simulink model "Ahmad_Ro"  (R2025b)
settings: Solver=VariableStepAuto  StartTime=0.0  StopTime=10.0  RelTol=1e-3
undefined symbols (not defined in the file or in its folder): X, Y, Z
libraries: sm_lib x16, nesl_utility x5, robotcorelib x1, robotmaniplib x1
settings Model: Creator=Ahmad Hz  LastModifiedBy=Ahmad Hz
settings ExplorerConfigSet: InternalSimMechanicsExplorerSettings=|
  | <ExplorerConfiguration>
  | 
  |   <canonicalview>default</canonicalview>
  | 
  |   <TilePanel>
  |     <TileInfo>
  |       <Tiles Columns="1" Count="1" Height="498" Rows="1" Width="971">
  |         <Row Weight="1"/>
  |         <Column Weight="1"/>
  |         <Tile Height="1" Width="1" X="0" Y="0"/>
  |       </Tiles>
  |     </TileInfo>
  |     <SceneInfo>
  |       <SceneViewer>
  |         <IsThisViewStd>
  |           <IsStandardView>off</IsStandardView>
  |           <StandardViewName>Front</StandardViewName>
  |         </IsThisViewStd>
  |         <BGColor>
  |           <R>1</R>
  |           <G>1</G>
  |           <B>1</B>
  |           <A>1</A>
  |         </BGColor>
  |         <Camera>
  |           <DoPerspective>off</DoPerspective>
  |           <Position>
  |             <X>0.69878161416282247</X>
  |             <Y>-0.56958841515750935</Y>
  |             <Z>0.67013251417587816</Z>
  |           </Position>
  |           <Center>
  |             <X>0.088649099502656606</X>
  |             <Y>0.040544099502656611</Y>
  |             <Z>0.059999999515712263</Z>
  |           </Center>
  |           <Up>
  |             <X>-0.40824829046386313</X>
  |             <Y>0.40824829046386302</Y>
  |             <Z>0.81649658092772603</Z>
  |           </Up>
  |           <XLim>0.14683425317748552</XLim>
  |           <YLim>0.14683425317748552</YLim>
  |           <ViewLimDist>0.01</ViewLimDist>
  |         </Camera>
  |       </SceneViewer>
  |     </SceneInfo>
  |   </TilePanel>
  | 
  |   <MechEditorPanel>
  |     <GfxPanelCameraMap/>
  |     <Cameras/>
  |     <VideoCreator>
  |       <IncludeTiles>All</IncludeTiles>
  |       <IncludeTime>on</IncludeTime>
  |       <IncludeWorldFrame>off</IncludeWorldFrame>
  |       <PlaybackSpeedRatio>1</PlaybackSpeedRatio>
  |       <FrameRate>30</FrameRate>
  |       <FrameSize>auto</FrameSize>
  |       <VideoFormat>MotionJPEGAVI</VideoFormat>
  |     </VideoCreator>
  |   </MechEditorPanel>
  | 
  |   <PlaybackSettings>
  |     <PlaybackSpeedFactor>1</PlaybackSpeedFactor>
  |   </PlaybackSettings>
  | 
  | </ExplorerConfiguration>

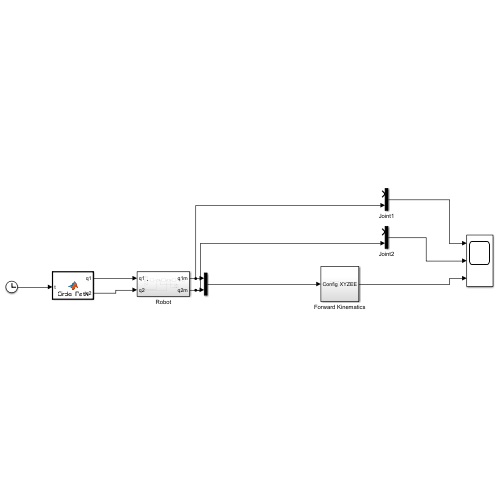
[thumbnail: Simulink's stored preview of the top-level diagram]
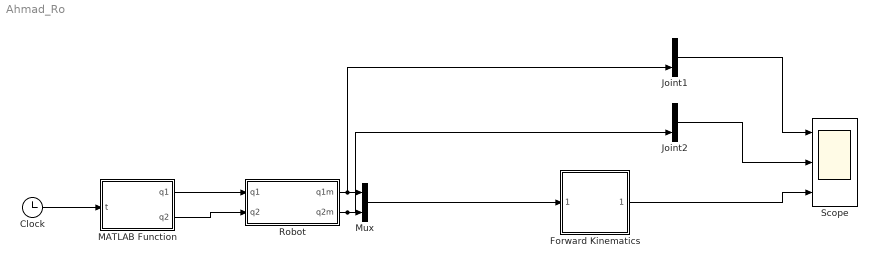
== system Ahmad_Ro ==
  Clock : Clock
  Forward Kinematics : Subsystem
  Joint1 : Mux  Inputs=2
  Joint2 : Mux  Inputs=2
  MATLAB Function : MATLAB Function  TreatAsAtomicUnit=on
  Mux : Mux  Inputs=2
  Robot : Subsystem
  Scope : Scope  NumInputPorts=3
      settings: ActiveDisplayYMinimum=-2.7504115188527223  ActiveDisplayYMaximum=3.3779479158130368
  wires:
  Robot/1(q1m) -> Joint1/2, Mux/1
  Robot/2(q2m) -> Joint2/2, Mux/2
  Joint1/1 -> Scope/1
  Joint2/1 -> Scope/2
  Mux/1 -> Forward Kinematics/1(Config)
  Forward Kinematics/1(XYZEE) -> Scope/3
  MATLAB Function/1(q1) -> Robot/1(q1)
  MATLAB Function/2(q2) -> Robot/2(q2)
  Clock/1 -> MATLAB Function/1(t)

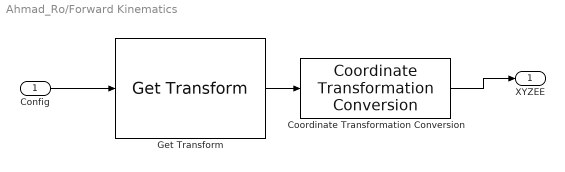
== system Ahmad_Ro/Forward Kinematics ==
  Config : Inport
  Coordinate Transformation Conversion : robotcorelib/Coordinate Transformation Conversion  InputRepresentation=Homogeneous Transformation  InputEulerSequence=ZYX  ShowTrVecInputPort=on  OutputRepresentation=Translation Vector  OutputEulerSequence=ZYX  ShowTrVecOutputPort=on  SimulateUsing=Interpreted execution
  Get Transform : robotmaniplib/Get Transform  RigidBodyTree=twoJointRigidBodyTree  SourceBody=tool  TargetBody=base  SimulateUsing=Interpreted execution
  XYZEE : Outport
  wires:
  Get Transform/1 -> Coordinate Transformation Conversion/1
  Coordinate Transformation Conversion/1 -> XYZEE/1
  Config/1 -> Get Transform/1

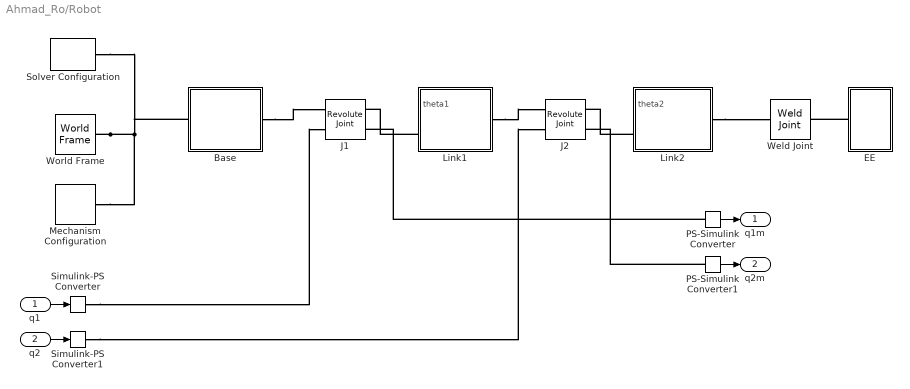
== system Ahmad_Ro/Robot ==
  q1 : Inport
  q2 : Inport  Port=2
  Base : Subsystem
  EE : Subsystem
  J1 : sm_lib/Joints/Revolute Joint  JointMode=Normal  CompositeWrenchDir=FollowerOnBase  CompositeWrenchFrame=BaseFrame  SenseConstraintForce=off  SenseConstraintTorque=off  SenseTotalForce=off  SenseTotalTorque=off  PositionTargetSpecify=off  PositionTargetPriority=High  PositionTargetValue=0  PositionTargetValueUnits=deg  VelocityTargetSpecify=off  VelocityTargetPriority=High  VelocityTargetValue=0  VelocityTargetValueUnits=deg/s  EquilibriumPosition=0  EquilibriumPositionUnits=deg  SpringStiffness=0  SpringStiffnessUnits=N*m/deg  DampingCoefficient=0  DampingCoefficientUnits=N*m/(deg/s)  LowerLimitSpecify=on  LowerLimitBound=-90  LowerLimitBoundUnits=deg  LowerLimitStiffness=1e4  LowerLimitStiffnessUnits=N*m/deg  LowerLimitDamping=10  LowerLimitDampingUnits=N*m/(deg/s)  LowerLimitTransitionRegionWidth=0.1  LowerLimitTransitionRegionWidthUnits=deg  UpperLimitSpecify=on  UpperLimitBound=90  UpperLimitBoundUnits=deg  UpperLimitStiffness=1e4  UpperLimitStiffnessUnits=N*m/deg  UpperLimitDamping=10  UpperLimitDampingUnits=N*m/(deg/s)  UpperLimitTransitionRegionWidth=0.1  UpperLimitTransitionRegionWidthUnits=deg  TorqueActuationMode=ComputedTorque  MotionActuationMode=InputMotion  SensePosition=on  SenseVelocity=off  SenseAcceleration=off  SenseTorqueForce=off  SenseLowerLimitTorqueForce=off  SenseUpperLimitTorqueForce=off
  J2 : sm_lib/Joints/Revolute Joint  JointMode=Normal  CompositeWrenchDir=FollowerOnBase  CompositeWrenchFrame=BaseFrame  SenseConstraintForce=off  SenseConstraintTorque=off  SenseTotalForce=off  SenseTotalTorque=off  PositionTargetSpecify=off  PositionTargetPriority=High  PositionTargetValue=0  PositionTargetValueUnits=deg  VelocityTargetSpecify=off  VelocityTargetPriority=High  VelocityTargetValue=0  VelocityTargetValueUnits=deg/s  EquilibriumPosition=0  EquilibriumPositionUnits=deg  SpringStiffness=0  SpringStiffnessUnits=N*m/deg  DampingCoefficient=0  DampingCoefficientUnits=N*m/(deg/s)  LowerLimitSpecify=on  LowerLimitBound=-60  LowerLimitBoundUnits=deg  LowerLimitStiffness=1e4  LowerLimitStiffnessUnits=N*m/deg  LowerLimitDamping=10  LowerLimitDampingUnits=N*m/(deg/s)  LowerLimitTransitionRegionWidth=0.1  LowerLimitTransitionRegionWidthUnits=deg  UpperLimitSpecify=on  UpperLimitBound=60  UpperLimitBoundUnits=deg  UpperLimitStiffness=1e4  UpperLimitStiffnessUnits=N*m/deg  UpperLimitDamping=10  UpperLimitDampingUnits=N*m/(deg/s)  UpperLimitTransitionRegionWidth=0.1  UpperLimitTransitionRegionWidthUnits=deg  TorqueActuationMode=ComputedTorque  MotionActuationMode=InputMotion  SensePosition=on  SenseVelocity=off  SenseAcceleration=off  SenseTorqueForce=off  SenseLowerLimitTorqueForce=off  SenseUpperLimitTorqueForce=off
  Link1 : Subsystem
  Link2 : Subsystem
  Mechanism Configuration : sm_lib/Utilities/Mechanism Configuration  UniformGravity=Constant  GravityVector=[0 0 -9.80665]  GravityVectorUnits=m/s^2  LinearizationDelta=0.001  JointModeTransitionNonlinearIterations=2
  PS-Simulink Converter : nesl_utility/PS-Simulink Converter  PhysicalDomain=network_engine_domain  SubClassName=ps_output  LeftPortType=input  RightPortType=output  PseudoPeriodic=off  Frequencies=[]  VectorFormat=inherit  Unit=inherit  AffineConversion=off
  PS-Simulink Converter1 : nesl_utility/PS-Simulink Converter  PhysicalDomain=network_engine_domain  SubClassName=ps_output  LeftPortType=input  RightPortType=output  PseudoPeriodic=off  Frequencies=[]  VectorFormat=inherit  Unit=inherit  AffineConversion=off
  Simulink-PS Converter : nesl_utility/Simulink-PS Converter  PhysicalDomain=network_engine_domain  SubClassName=ps_input  LeftPortType=input  RightPortType=output  PseudoPeriodic=off  Frequencies=[]  NoiseDistribution=none  NoiseParameters=[]  Unit=rad  AffineConversion=off  FilteringAndDerivatives=filter  SimscapeFilterOrder=2  InputFilterTimeConstant=0.001  UdotUserProvided=0
  Simulink-PS Converter1 : nesl_utility/Simulink-PS Converter  PhysicalDomain=network_engine_domain  SubClassName=ps_input  LeftPortType=input  RightPortType=output  PseudoPeriodic=off  Frequencies=[]  NoiseDistribution=none  NoiseParameters=[]  Unit=rad  AffineConversion=off  FilteringAndDerivatives=filter  SimscapeFilterOrder=2  InputFilterTimeConstant=0.001  UdotUserProvided=0
  Solver Configuration : nesl_utility/Solver Configuration  PhysicalDomain=network_engine_domain  SubClassName=solver  LeftPortType=input  RightPortType=generic  Tones=[]  Harmonics=[]  SimulateNoise=off  Profile=off  UseLocalSampling=off  EnableSwitchedLinearOptims=on  FrequencyDomain=off  UseCCode=off  RelTol=0.001  AbsTol=0.001  MinStep=1e-09  ToWorkspace=off  RevertToSquareIcSolve=off  NumHomotopyIterations=100  PhasorMode=off  PhasorModeNumHarmonics=1  ConsistencySolver=NEWTON_XTOL_AFTER_FTOL  IndexReductionMethod=DerivativeReplacement  DoDC=off  ResidualTolerance=1e-09  ConsistencyTolSource=GLOBAL  ConsistencyAbsTol=0.001  ConsistencyRelTol=0.001  ConsistencyTolFactor=0.001  UseLocalSolver=off  LocalSolverChoice=NE_BACKWARD_EULER_ADVANCER  ResolveIndetEquations=on  FunctionEvalNumThread=1  LocalSolverSampleTime=0.001  DoFixedCost=off  MaxNonlinIter=3  MaxModeIter=2  ComputeImpulses=off  ImpulseIterations=2  LinearAlgebra=auto  LinearAlgebraNumThread=0  EquationFormulation=NE_TIME_EF  DelaysMemoryBudget=1024  AutomaticFiltering=on  FilteringTimeConstant=0.001  PartitionStorageMethod=AS_NEEDED  PartitionMemoryBudget=1024  PartitionMethod=ROBUST  MultibodyUseLocalSolver=off  MultibodyLocalSolverChoice=ODE1  MultibodyLocalSolverSampleTime=0.001
  Weld Joint : sm_lib/Joints/Weld Joint  JointMode=Normal  CompositeWrenchDir=FollowerOnBase  CompositeWrenchFrame=BaseFrame  SenseConstraintForce=off  SenseConstraintTorque=off  SenseTotalForce=off  SenseTotalTorque=off
  World Frame : sm_lib/Frames and Transforms/World Frame
  q1m : Outport
  q2m : Outport  Port=2
  wires:
  q2/1 -> Simulink-PS Converter1/1
  PS-Simulink Converter/1 -> q1m/1
  q1/1 -> Simulink-PS Converter/1
  PS-Simulink Converter1/1 -> q2m/1
  connections:
  Link1/LConn1 -- J1/RConn1
  EE/LConn1 -- Weld Joint/RConn1
  World Frame/RConn1 -- Solver Configuration/RConn1 -- Base/LConn1 -- Mechanism Configuration/RConn1
  PS-Simulink Converter1/LConn1 -- J2/RConn2
  Simulink-PS Converter1/RConn1 -- J2/LConn2
  PS-Simulink Converter/LConn1 -- J1/RConn2
  Link1/RConn1 -- J2/LConn1
  Base/RConn1 -- J1/LConn1
  Link2/RConn1 -- Weld Joint/LConn1
  Link2/LConn1 -- J2/RConn1
  Simulink-PS Converter/RConn1 -- J1/LConn2

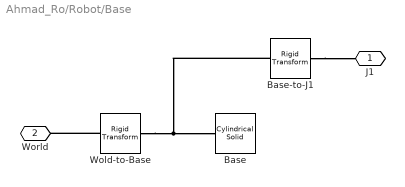
== system Ahmad_Ro/Robot/Base ==
  Base : sm_lib/Body Elements/Cylindrical Solid  CylinderRadius=0.05  CylinderRadiusUnits=m  CylinderLength=0.1  CylinderLengthUnits=m  ExportEntireGeometry=off  InertiaType=CalculateFromGeometry  BasedOnType=Density  Density=1000  DensityUnits=kg/m^3  Mass=1  MassUnits=kg  CenterOfMass=[0 0 0]  CenterOfMassUnits=m  MomentsOfInertia=[1 1 1]  MomentsOfInertiaUnits=kg*m^2  ProductsOfInertia=[0 0 0]  ProductsOfInertiaUnits=kg*m^2  GraphicType=FromGeometry  MarkerShape=Sphere  MarkerSize=10  GraphicVisPropType=SimpleVisualProperties  GraphicDiffuseColor=[0 0 1]  GraphicOpacity=1  GraphicSpecularColor=[0.5 0.5 0.5 1.0]  GraphicAmbientColor=[0.15 0.15 0.15 1.0]  GraphicEmissiveColor=[0.0 0.0 0.0 1.0]  GraphicShininess=75  DoExposeReferenceFrame=on  SerializedFrames=<Frames/>
  Base-to-J1 : sm_lib/Frames and Transforms/Rigid Transform  RotationMethod=None  FollAlignAxisA=+X  BaseAlignAxisA=+Y  FollAlignAxisB=+Y  BaseAlignAxisB=+Z  RotationStandardAxis=+Z  RotationAngle=0  RotationAngleUnits=deg  RotationArbitraryAxis=[0 0 1]  RotationSequenceAxes=FollowerAxes  RotationSequence=XYX  RotationSequenceAngles=[0 0 0]  RotationSequenceAnglesUnits=deg  RotationMatrix=[1 0 0;0 1 0;0 0 1]  Quaternion=[1 0 0 0]  TranslationMethod=Cartesian  TranslationCartesianOffset=[0 0 0.06]  TranslationCartesianOffsetUnits=m  TranslationStandardAxis=+Z  TranslationStandardOffset=0  TranslationStandardOffsetUnits=m  TranslationROffset=0  TranslationROffsetUnits=m  TranslationThetaOffset=0  TranslationThetaOffsetUnits=deg  TranslationZOffset=0  TranslationZOffsetUnits=m
  Wold-to-Base : sm_lib/Frames and Transforms/Rigid Transform  RotationMethod=None  FollAlignAxisA=+X  BaseAlignAxisA=+Y  FollAlignAxisB=+Y  BaseAlignAxisB=+Z  RotationStandardAxis=+Z  RotationAngle=0  RotationAngleUnits=deg  RotationArbitraryAxis=[0 0 1]  RotationSequenceAxes=FollowerAxes  RotationSequence=XYX  RotationSequenceAngles=[0 0 0]  RotationSequenceAnglesUnits=deg  RotationMatrix=[1 0 0;0 1 0;0 0 1]  Quaternion=[1 0 0 0]  TranslationMethod=Cartesian  TranslationCartesianOffset=[0 0 0.05]  TranslationCartesianOffsetUnits=m  TranslationStandardAxis=+Z  TranslationStandardOffset=0  TranslationStandardOffsetUnits=m  TranslationROffset=0  TranslationROffsetUnits=m  TranslationThetaOffset=0  TranslationThetaOffsetUnits=deg  TranslationZOffset=0  TranslationZOffsetUnits=m
  J1 : PMIOPort  Side=Right
  World : PMIOPort  Port=2  Side=Left
  connections:
  Wold-to-Base/RConn1 -- Base-to-J1/LConn1 -- Base/RConn1
  Wold-to-Base/LConn1 -- World/RConn1
  Base-to-J1/RConn1 -- J1/RConn1

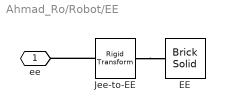
== system Ahmad_Ro/Robot/EE ==
  EE : sm_lib/Body Elements/Brick Solid  BrickDimensions=[0.02 0.02 0.02]  BrickDimensionsUnits=m  ExportEntireGeometry=off  InertiaType=CalculateFromGeometry  BasedOnType=Density  Density=1000  DensityUnits=kg/m^3  Mass=1  MassUnits=kg  CenterOfMass=[0 0 0]  CenterOfMassUnits=m  MomentsOfInertia=[1 1 1]  MomentsOfInertiaUnits=kg*m^2  ProductsOfInertia=[0 0 0]  ProductsOfInertiaUnits=kg*m^2  GraphicType=FromGeometry  MarkerShape=Sphere  MarkerSize=10  GraphicVisPropType=SimpleVisualProperties  GraphicDiffuseColor=[0 0 0]  GraphicOpacity=1  GraphicSpecularColor=[0.5 0.5 0.5 1.0]  GraphicAmbientColor=[0.15 0.15 0.15 1.0]  GraphicEmissiveColor=[0.0 0.0 0.0 1.0]  GraphicShininess=75  DoExposeReferenceFrame=on  SerializedFrames=<Frames/>
  Jee-to-EE : sm_lib/Frames and Transforms/Rigid Transform  RotationMethod=None  FollAlignAxisA=+X  BaseAlignAxisA=+Y  FollAlignAxisB=+Y  BaseAlignAxisB=+Z  RotationStandardAxis=+Z  RotationAngle=0  RotationAngleUnits=deg  RotationArbitraryAxis=[0 0 1]  RotationSequenceAxes=FollowerAxes  RotationSequence=XYX  RotationSequenceAngles=[0 0 0]  RotationSequenceAnglesUnits=deg  RotationMatrix=[1 0 0;0 1 0;0 0 1]  Quaternion=[1 0 0 0]  TranslationMethod=Cartesian  TranslationCartesianOffset=[0.01 0 0]  TranslationCartesianOffsetUnits=m  TranslationStandardAxis=+Z  TranslationStandardOffset=0  TranslationStandardOffsetUnits=m  TranslationROffset=0  TranslationROffsetUnits=m  TranslationThetaOffset=0  TranslationThetaOffsetUnits=deg  TranslationZOffset=0  TranslationZOffsetUnits=m
  ee : PMIOPort  Side=Left
  connections:
  Jee-to-EE/RConn1 -- EE/RConn1
  Jee-to-EE/LConn1 -- ee/RConn1

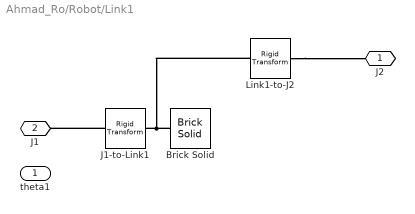
== system Ahmad_Ro/Robot/Link1 ==
  theta1 : Inport
  Brick Solid : sm_lib/Body Elements/Brick Solid  BrickDimensions=[0.2 0.02 0.02]  BrickDimensionsUnits=m  ExportEntireGeometry=off  InertiaType=CalculateFromGeometry  BasedOnType=Density  Density=1000  DensityUnits=kg/m^3  Mass=1  MassUnits=kg  CenterOfMass=[0 0 0]  CenterOfMassUnits=m  MomentsOfInertia=[1 1 1]  MomentsOfInertiaUnits=kg*m^2  ProductsOfInertia=[0 0 0]  ProductsOfInertiaUnits=kg*m^2  GraphicType=FromGeometry  MarkerShape=Sphere  MarkerSize=10  GraphicVisPropType=SimpleVisualProperties  GraphicDiffuseColor=[0 1 0.498]  GraphicOpacity=1  GraphicSpecularColor=[0.5 0.5 0.5 1.0]  GraphicAmbientColor=[0.15 0.15 0.15 1.0]  GraphicEmissiveColor=[0.0 0.0 0.0 1.0]  GraphicShininess=75  DoExposeReferenceFrame=on  SerializedFrames=<Frames/>
  J1-to-Link1 : sm_lib/Frames and Transforms/Rigid Transform  RotationMethod=None  FollAlignAxisA=+X  BaseAlignAxisA=+Y  FollAlignAxisB=+Y  BaseAlignAxisB=+Z  RotationStandardAxis=+Z  RotationAngle=0  RotationAngleUnits=deg  RotationArbitraryAxis=[0 0 1]  RotationSequenceAxes=FollowerAxes  RotationSequence=XYX  RotationSequenceAngles=[0 0 0]  RotationSequenceAnglesUnits=deg  RotationMatrix=[1 0 0;0 1 0;0 0 1]  Quaternion=[1 0 0 0]  TranslationMethod=Cartesian  TranslationCartesianOffset=[0.1 0 0]  TranslationCartesianOffsetUnits=m  TranslationStandardAxis=+Z  TranslationStandardOffset=0  TranslationStandardOffsetUnits=m  TranslationROffset=0  TranslationROffsetUnits=m  TranslationThetaOffset=0  TranslationThetaOffsetUnits=deg  TranslationZOffset=0  TranslationZOffsetUnits=m
  Link1-to-J2 : sm_lib/Frames and Transforms/Rigid Transform  RotationMethod=None  FollAlignAxisA=+X  BaseAlignAxisA=+Y  FollAlignAxisB=+Y  BaseAlignAxisB=+Z  RotationStandardAxis=+Z  RotationAngle=0  RotationAngleUnits=deg  RotationArbitraryAxis=[0 0 1]  RotationSequenceAxes=FollowerAxes  RotationSequence=XYX  RotationSequenceAngles=[0 0 0]  RotationSequenceAnglesUnits=deg  RotationMatrix=[1 0 0;0 1 0;0 0 1]  Quaternion=[1 0 0 0]  TranslationMethod=Cartesian  TranslationCartesianOffset=[0.1 0 0]  TranslationCartesianOffsetUnits=m  TranslationStandardAxis=+Z  TranslationStandardOffset=0  TranslationStandardOffsetUnits=m  TranslationROffset=0  TranslationROffsetUnits=m  TranslationThetaOffset=0  TranslationThetaOffsetUnits=deg  TranslationZOffset=0  TranslationZOffsetUnits=m
  J2 : PMIOPort  Side=Right
  J1 : PMIOPort  Port=2  Side=Left
  connections:
  Brick Solid/RConn1 -- Link1-to-J2/LConn1 -- J1-to-Link1/RConn1
  J1-to-Link1/LConn1 -- J1/RConn1
  Link1-to-J2/RConn1 -- J2/RConn1

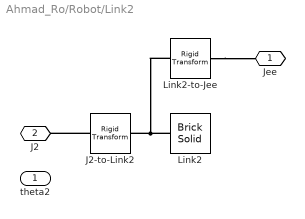
== system Ahmad_Ro/Robot/Link2 ==
  theta2 : Inport
  J2-to-Link2 : sm_lib/Frames and Transforms/Rigid Transform  RotationMethod=None  FollAlignAxisA=+X  BaseAlignAxisA=+Y  FollAlignAxisB=+Y  BaseAlignAxisB=+Z  RotationStandardAxis=+Z  RotationAngle=0  RotationAngleUnits=deg  RotationArbitraryAxis=[0 0 1]  RotationSequenceAxes=FollowerAxes  RotationSequence=XYX  RotationSequenceAngles=[0 0 0]  RotationSequenceAnglesUnits=deg  RotationMatrix=[1 0 0;0 1 0;0 0 1]  Quaternion=[1 0 0 0]  TranslationMethod=Cartesian  TranslationCartesianOffset=[0.075 0 0]  TranslationCartesianOffsetUnits=m  TranslationStandardAxis=+Z  TranslationStandardOffset=0  TranslationStandardOffsetUnits=m  TranslationROffset=0  TranslationROffsetUnits=m  TranslationThetaOffset=0  TranslationThetaOffsetUnits=deg  TranslationZOffset=0  TranslationZOffsetUnits=m
  Link2 : sm_lib/Body Elements/Brick Solid  BrickDimensions=[0.15 0.02 0.02]  BrickDimensionsUnits=m  ExportEntireGeometry=off  InertiaType=CalculateFromGeometry  BasedOnType=Density  Density=1000  DensityUnits=kg/m^3  Mass=1  MassUnits=kg  CenterOfMass=[0 0 0]  CenterOfMassUnits=m  MomentsOfInertia=[1 1 1]  MomentsOfInertiaUnits=kg*m^2  ProductsOfInertia=[0 0 0]  ProductsOfInertiaUnits=kg*m^2  GraphicType=FromGeometry  MarkerShape=Sphere  MarkerSize=10  GraphicVisPropType=SimpleVisualProperties  GraphicDiffuseColor=[0.6667 0 1]  GraphicOpacity=1  GraphicSpecularColor=[0.5 0.5 0.5 1.0]  GraphicAmbientColor=[0.15 0.15 0.15 1.0]  GraphicEmissiveColor=[0.0 0.0 0.0 1.0]  GraphicShininess=75  DoExposeReferenceFrame=on  SerializedFrames=<Frames/>
  Link2-to-Jee : sm_lib/Frames and Transforms/Rigid Transform  RotationMethod=None  FollAlignAxisA=+X  BaseAlignAxisA=+Y  FollAlignAxisB=+Y  BaseAlignAxisB=+Z  RotationStandardAxis=+Z  RotationAngle=0  RotationAngleUnits=deg  RotationArbitraryAxis=[0 0 1]  RotationSequenceAxes=FollowerAxes  RotationSequence=XYX  RotationSequenceAngles=[0 0 0]  RotationSequenceAnglesUnits=deg  RotationMatrix=[1 0 0;0 1 0;0 0 1]  Quaternion=[1 0 0 0]  TranslationMethod=Cartesian  TranslationCartesianOffset=[0.075 0 0]  TranslationCartesianOffsetUnits=m  TranslationStandardAxis=+Z  TranslationStandardOffset=0  TranslationStandardOffsetUnits=m  TranslationROffset=0  TranslationROffsetUnits=m  TranslationThetaOffset=0  TranslationThetaOffsetUnits=deg  TranslationZOffset=0  TranslationZOffsetUnits=m
  Jee : PMIOPort  Side=Right
  J2 : PMIOPort  Port=2  Side=Left
  connections:
  J2-to-Link2/LConn1 -- J2/RConn1
  Link2/RConn1 -- Link2-to-Jee/LConn1 -- J2-to-Link2/RConn1
  Link2-to-Jee/RConn1 -- Jee/RConn1

== matlab function Ahmad_Ro/MATLAB Function ==
  data: t input; q1 output; q2 output
function [q1, q2] = Square_Controller(t)
    L1 = 0.2; L2 = 0.15;
    
    T = 10;
    phase = mod(t, T);
    
    P1 = [0.15, 0.01]; P2 = [0.25, 0.01];
    P3 = [0.25, 0.11]; P4 = [0.15, 0.11];
    
    if phase < T/4
        target = P1 + (P2-P1)*(phase/(T/4));
    elseif phase < T/2
        target = P2 + (P3-P2)*((phase-T/4)/(T/4));
    elseif phase < 3*T/4
        target = P3 + (P4-P3)*((phase-T/2)/(T/4));
    else
        target = P4 + (P1-P4)*((phase-3*T/4)/(T/4));
    end
    
    x = target(1); y = target(2);

    cos_q2 = (x^2 + y^2 - L1^2 - L2^2) / (2 * L1 * L2);
    q2 = acos(cos_q2);
    q1 = atan2(y, x) - atan2(L2*sin(q2), L1 + L2*cos(q2));
end
